simulink model "final"  (R2026a)
settings: Solver=VariableStepAuto  StopTime=10000
libraries: simulink x4
settings Model: Creator=humpr  LastModifiedBy=humpr

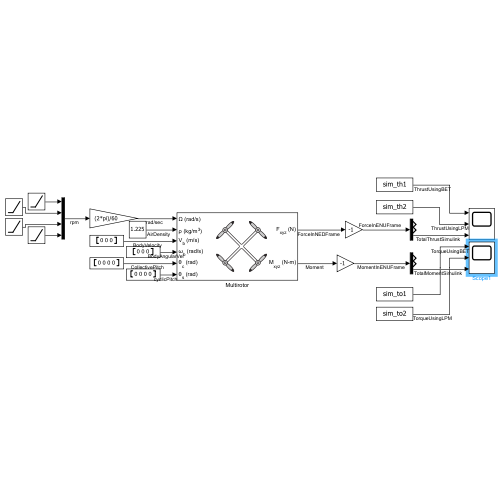
[thumbnail: Simulink's stored preview of the top-level diagram]
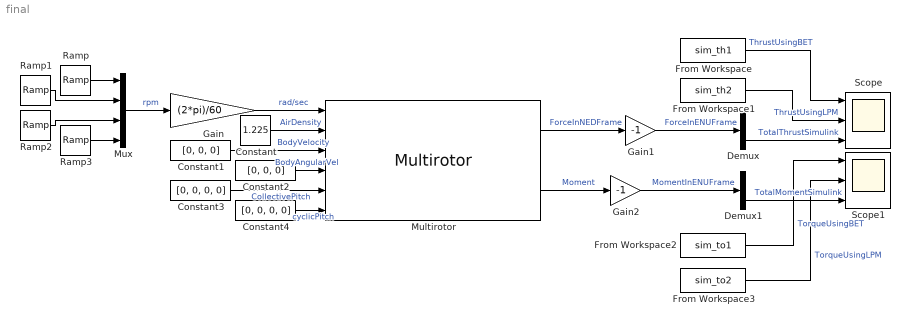
== system final ==
  Constant : Constant  Value=1.225
  Constant1 : Constant  Value=[0, 0, 0]
  Constant2 : Constant  Value=[0, 0, 0]
  Constant3 : Constant  Value=[0, 0, 0, 0]
  Constant4 : Constant  Value=[0, 0, 0, 0]
  Demux : Demux  Outputs=3
  Demux1 : Demux  Outputs=3
  From Workspace : FromWorkspace  VariableName=sim_th1
  From Workspace1 : FromWorkspace  VariableName=sim_th2
  From Workspace2 : FromWorkspace  VariableName=sim_to1
  From Workspace3 : FromWorkspace  VariableName=sim_to2
  Gain : Gain  Gain=(2*pi)/60
  Gain1 : Gain  Gain=-1
  Gain2 : Gain  Gain=-1
  Multirotor : Multirotor  modelMode=With flap effects  controlInput=on  CT=0.0315  CQ=0.0089  radius=(5/2)*0.0254  chord=0.015  hingeOffset=0.005  clalpha=2*pi  thetaRoot=30*pi/180  thetaTwist=(5-30)*pi/180
  Mux : Mux
  Ramp{,1..3} (4 alike) : simulink/Sources/Ramp  slope=1  start=0  InitialOutput=0
  Scope : Scope  NumInputPorts=3
      settings: ActiveDisplayYMinimum=-0.2700950399163432  ActiveDisplayYMaximum=2.4308553592470892
  Scope1 : Scope  NumInputPorts=3
      settings: ActiveDisplayYMinimum=-0.0048531983667012366  ActiveDisplayYMaximum=0.043678785300311135
  wires:
  Ramp1/1 -> Mux/2
  Ramp2/1 -> Mux/3
  Ramp/1 -> Mux/1
  Ramp3/1 -> Mux/4
  Mux/1 -> Gain/1  "rpm"
  Gain/1 -> Multirotor/1  "rad/sec"
  Constant/1 -> Multirotor/2  "AirDensity"
  Constant1/1 -> Multirotor/3  "BodyVelocity"
  Constant2/1 -> Multirotor/4  "BodyAngularVel"
  Constant3/1 -> Multirotor/5  "CollectivePitch"
  Constant4/1 -> Multirotor/6  "cyclicPitch"
  Multirotor/1 -> Gain1/1  "ForceInNEDFrame"
  Multirotor/2 -> Gain2/1  "Moment"
  Gain1/1 -> Demux/1  "ForceInENUFrame"
  Gain2/1 -> Demux1/1  "MomentInENUFrame"
  Demux1/3 -> Scope1/3  "TotalMomentSimulink"
  Demux/3 -> Scope/3  "TotalThrustSimulink"
  From Workspace/1 -> Scope/1  "ThrustUsingBET"
  From Workspace1/1 -> Scope/2  "ThrustUsingLPM"
  From Workspace2/1 -> Scope1/1  "TorqueUsingBET"
  From Workspace3/1 -> Scope1/2  "TorqueUsingLPM"
